simulink model "Six_Step"  (R2023a)
settings: Solver=FixedStepDiscrete  StartTime=0.0  StopTime=SC.T  FixedStep=P.dt  RelTol=1e-3
PreLoadFcn:
  | d_ = fileparts(get_param(bdroot,'FileName')); addpath(d_, fullfile(d_, '..', 'Common')); clear d_; six_step_init;
values from neighbouring files (symbols this model uses):
  DECIM = 10    [six_step_init.m]
  P = bldc_params()    [six_step_init.m]
  SS = struct()    [six_step_init.m]
undefined symbols (not defined in the file or in its folder): THETA_OFF
libraries: bldc_plant_lib x5, slpidlib x2, spspowerguiLib x1
settings Model: Creator=PC  LastModifiedBy=PC

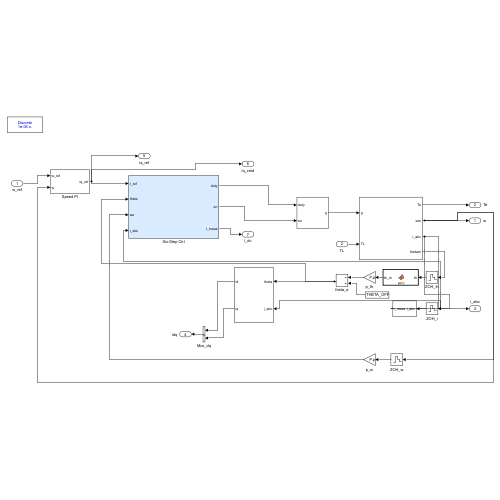
[thumbnail: Simulink's stored preview of the top-level diagram]
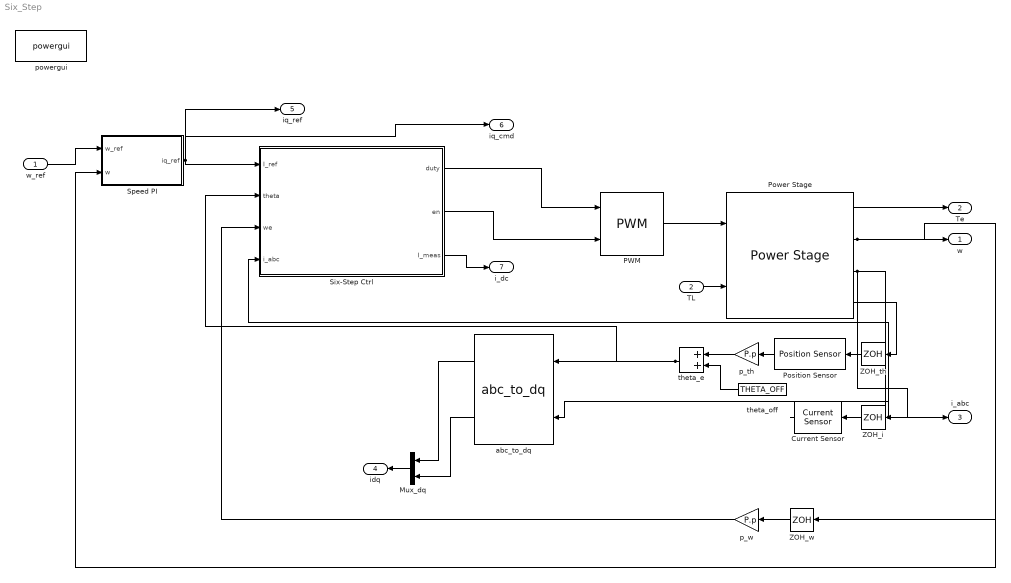
== system Six_Step ==
  w_ref : Inport  Interpolate=off
  TL : Inport  Port=2  Interpolate=off
  Current Sensor : bldc_plant_lib/Current Sensor  Description=Phase-current sensors: i_meas = P.CS.M*(P.CS.gain.*i_abc + P.CS.off). Ideal by default (bldc_set_sensor).  SystemSampleTime=-1  VariantActivationTime=update diagram  Latency=0  AutoFrameSizeCalculation=off
  Mux_dq : Mux  Inputs=2
  PWM : bldc_plant_lib/PWM  SystemSampleTime=-1  VariantActivationTime=update diagram  Latency=0  AutoFrameSizeCalculation=off
  Position Sensor : bldc_plant_lib/Position Sensor  Description=Position sensor: quantized mechanical angle + mounting offset (P.ENC, bldc_set_encoder). Ideal by default.  SystemSampleTime=-1  VariantActivationTime=update diagram  Latency=0  AutoFrameSizeCalculation=off
      settings: LibrarySourceBlock=|
      | simulink/User-Defined
      | Functions/MATLAB Function
  Power Stage : bldc_plant_lib/Power Stage  SystemSampleTime=-1  VariantActivationTime=update diagram  Latency=0  AutoFrameSizeCalculation=off
  Six-Step Ctrl : Subsystem
  Speed PI : Subsystem
  ZOH_i : ZeroOrderHold  SampleTime=P.Ts
  ZOH_th : ZeroOrderHold  SampleTime=P.Ts
  ZOH_w : ZeroOrderHold  SampleTime=P.Ts
  abc_to_dq : bldc_plant_lib/abc_to_dq  SystemSampleTime=-1  VariantActivationTime=update diagram  Latency=0  AutoFrameSizeCalculation=off
  p_th : Gain  Gain=P.p
  p_w : Gain  Gain=P.p
  powergui : spspowerguiLib/powergui  Priority=1  SimulationMode=Discrete  SampleTime=P.dt  frequency=60  Iterations=50  frequencyindice=0  Pbase=100e6  ErrMax=1e-4  UnitsV=kV  UnitsW=MW  buscounter=0  FunctionMessages=off  echomessages=off  EnableUseOfTLC=off  CurrentSourceSwitches=off  DisableSnubberDevices=off  DisableRonSwitches=off  DisableVfSwitches=off  DisplayEquations=off  AutomaticDiscreteSolvers=off  SolverType=Tustin/Backward Euler (TBE)  Interpol=off  ExternalGateDelay=off  methode=off  Ts=100  x0status=blocks  SPID=on  SwTol=0  HookPort=off  NonlinearTolerance=1e-4  nMaxIteration=100  ContinueOnMaxIteration=off  RestoreLinks=warning  ResistiveCurrentMeasurement=off  Frange=[0:2:500]  Ylog=off  Xlog=on  ShowGrid=off  save=off  variable=ZData  structure=0  ZoomFFT=off  StartTime=0.0  cycles=1  DisplayStyle=1  fundamental=60  FreqAxis=off  MaxFrequency=1000  frequencyindicesteady=1  RmsSteady=1  display=off
  theta_e : Sum
  theta_off : Constant  Value=THETA_OFF
  w : Outport  SampleTime=DECIM*P.dt
  Te : Outport  Port=2  SampleTime=DECIM*P.dt
  i_abc : Outport  Port=3  SampleTime=DECIM*P.dt
  idq : Outport  Port=4
  iq_ref : Outport  Port=5
  iq_cmd : Outport  Port=6
  i_dc : Outport  Port=7
  wires:
  w_ref/1 -> Speed PI/1(w_ref)
  Speed PI/1(iq_ref) -> iq_ref/1, Six-Step Ctrl/1(I_ref), iq_cmd/1
  TL/1 -> Power Stage/2
  PWM/1 -> Power Stage/1
  Power Stage/1 -> Te/1
  p_th/1 -> theta_e/1
  theta_off/1 -> theta_e/2
  ZOH_w/1 -> p_w/1
  abc_to_dq/1 -> Mux_dq/1
  abc_to_dq/2 -> Mux_dq/2
  Mux_dq/1 -> idq/1
  Six-Step Ctrl/1(duty) -> PWM/1
  Six-Step Ctrl/2(en) -> PWM/2
  Six-Step Ctrl/3(I_meas) -> i_dc/1
  Power Stage/2 -> w/1, ZOH_w/1, Speed PI/2(w)
  Power Stage/3 -> i_abc/1, ZOH_i/1
  Power Stage/4 -> ZOH_th/1
  theta_e/1 -> abc_to_dq/1, Six-Step Ctrl/2(theta)
  p_w/1 -> Six-Step Ctrl/3(we)
  ZOH_i/1 -> Current Sensor/1
  Current Sensor/1 -> abc_to_dq/2, Six-Step Ctrl/4(i_abc)
  ZOH_th/1 -> Position Sensor/1
  Position Sensor/1 -> p_th/1

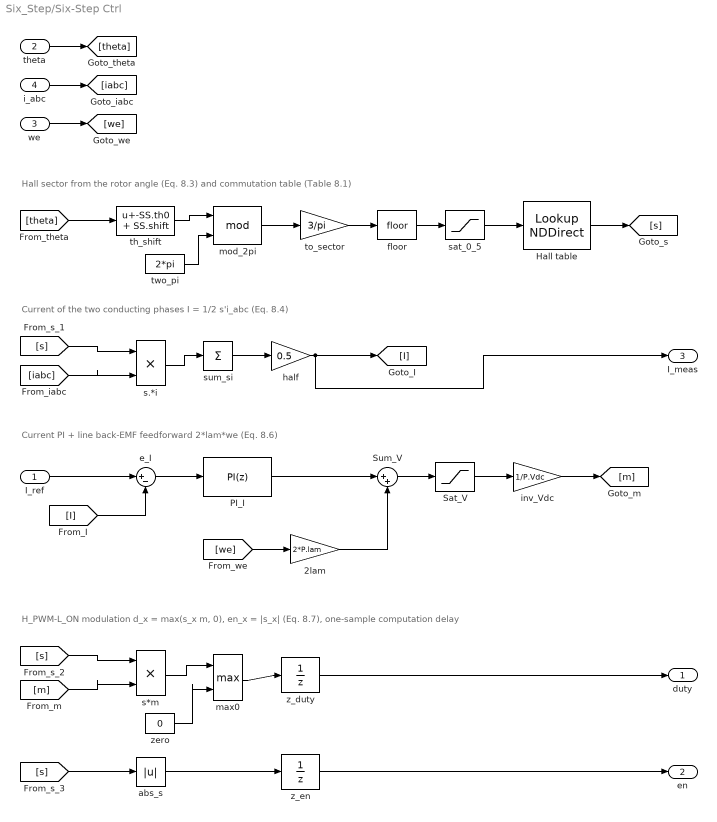
== system Six_Step/Six-Step Ctrl ==
  note: Hall sector from the rotor angle (Eq. 8.3) and commutation table (Table 8.1)
  note: Current of the two conducting phases I = 1/2 s'i_abc (Eq. 8.4)
  note: Current PI + line back-EMF feedforward 2*lam*we (Eq. 8.6)
  note: H_PWM-L_ON modulation d_x = max(s_x m, 0), en_x = |s_x| (Eq. 8.7), one-sample computation delay
  I_ref : Inport
  theta : Inport  Port=2
  we : Inport  Port=3
  i_abc : Inport  Port=4
  2lam : Gain  Gain=2*P.lam
  Hall table : LookupNDDirect  InputsSelectThisObjectFromTable=Vector  Table=SS.tab
  PI_I : slpidlib/PID Controller  Controller=PI  Form=Parallel  TimeDomain=Discrete-time  UseExternalTs=off  SampleTime=P.Ts  IntegratorMethod=Forward Euler  FilterMethod=Forward Euler  ControllerParametersSource=internal  P=P.Kp_i6  I=P.Ki_i6  UseKiTs=off  D=0  N=100  UseFilter=on  TunerSelectOption=Transfer Function Based (PID Tuner App)  InitialConditionSource=internal  InitialConditionForIntegrator=0  InitialConditionForFilter=0  DifferentiatorICPrevScaledInput=0  ExternalReset=none  TrackingMode=off  Kt=1  LimitOutput=on  SatLimitsSource=internal  UpperSaturationLimit=P.Vdc  LowerSaturationLimit=-P.Vdc  LinearizeAsGain=on  AntiWindupMode=back-calculation  Kb=(P.Ki_i6)/(P.Kp_i6)  LimitIntegrator=off  UpperIntegratorSaturationLimit=inf  LowerIntegratorSaturationLimit=-inf  POutMin=[]  POutMax=[]  IOutMin=[]  IOutMax=[]  DOutMin=[]  DOutMax=[]  NOutMin=[]  NOutMax=[]  SumOutMin=[]  SumOutMax=[]  SaturationOutMin=[]  SaturationOutMax=[]  PParamMin=[]  PParamMax=[]  IParamMin=[]  IParamMax=[]  DParamMin=[]  DParamMax=[]  NParamMin=[]  NParamMax=[]  KbParamMin=[]  KbParamMax=[]  KtParamMin=[]  KtParamMax=[]  KbOutMin=[]  KbOutMax=[]  KtOutMin=[]  KtOutMax=[]  IntegratorOutMin=[]  IntegratorOutMax=[]  FilterOutMin=[]  FilterOutMax=[]  SumI1OutMin=[]  SumI1OutMax=[]  SumI2OutMin=[]  SumI2OutMax=[]  SumI3OutMin=[]  SumI3OutMax=[]  SumI4OutMin=[]  SumI4OutMax=[]  SumDOutMin=[]  SumDOutMax=[]  DifferentiatorOutMin=[]  DifferentiatorOutMax=[]  FilterDiffOutCoefMin=[]  FilterDiffOutCoefMax=[]  ReciprocalOutMin=[]  ReciprocalOutMax=[]  SumDenOutMin=[]  SumDenOutMax=[]  SumNumOutMin=[]  SumNumOutMax=[]  DivideOutMin=[]  DivideOutMax=[]  UdiffTsProdOutMin=[]  UdiffTsProdOutMax=[]  NTsProdOutMin=[]  NTsProdOutMax=[]  UintegralTsProdOutMin=[]  UintegralTsProdOutMax=[]  UngainTsProdOutMin=[]  UngainTsProdOutMax=[]  ClampingZeroOutDataTypeStr=Inherit: Inherit via back propagation  ClampingZeroOutMin=[]  ClampingZeroOutMax=[]  FilterDenConstantOutDataTypeStr=Inherit: Inherit via back propagation  FilterDenConstantOutMin=[]  FilterDenConstantOutMax=[]  PCopyOutDataTypeStr=Inherit: Inherit via back propagation  PCopyOutMin=[]  PCopyOutMax=[]  NCopyOutDataTypeStr=Inherit: Inherit via back propagation  NCopyOutMin=[]  NCopyOutMax=[]  IntegratorContinuousStateAttributes=''  IntegratorStateMustResolveToSignalObject=off  IntegratorRTWStateStorageClass=Auto  FilterContinuousStateAttributes=''  FilterStateMustResolveToSignalObject=off  FilterRTWStateStorageClass=Auto  ParallelPVariant=InternalParameters  IdealPVariant=Disabled  IVariant=InternalParameters  DVariant=Disabled  IntegratorVariant=Discrete  SatVariant=Enabled  AWVariant=BackCalculation  PCopyVariant=Disabled  TRVariant=Disabled  FdbkBlocksVariant=Forward  IdealPFdbkVariant=Disabled  SatFdbkVariant=Disabled  DerivativeFilterVariant=Disabled  NVariant=Disabled  NCopyVariant=Disabled_SignalSpec  FilterICVariant=Disabled  IntegratorICVariant=InternalICs  ExternalResetVariant=Disabled  TRSumVariant=Passthrough  SumFdbkVariant=Disabled  SumVariant=Sum_PI  TsampFilterVariant=InternalTs  TsampNgainVariant=Passthrough  TsampIntegralVariant=Disabled_SignalSpec  ExternalSaturationOutDataTypeStr=Inherit: Same as second input
  Sat_V : Saturate  UpperLimit=P.Vdc  LowerLimit=-P.Vdc
  Sum_V : Sum  Inputs=|++
  abs_s : Abs
  e_I : Sum  Inputs=|+-
  floor : Rounding
  half : Gain  Gain=0.5
  inv_Vdc : Gain  Gain=1/P.Vdc
  max0 : MinMax  Function=max  Inputs=2
  mod_2pi : Math  Operator=mod
  s*m : Product
  s.*i : Product
  sat_0_5 : Saturate  UpperLimit=5  LowerLimit=0
  sum_si : Sum  Inputs=+
  th_shift : Bias  Bias=-SS.th0 + SS.shift
  to_sector : Gain  Gain=3/pi
  two_pi : Constant  Value=2*pi
  z_duty : UnitDelay  InitialCondition=zeros(3,1)  SampleTime=P.Ts
  z_en : UnitDelay  InitialCondition=zeros(3,1)  SampleTime=P.Ts
  zero : Constant  Value=0
  duty : Outport
  en : Outport  Port=2
  I_meas : Outport  Port=3
  wires:
  theta/1 -> [theta]
  i_abc/1 -> [iabc]
  we/1 -> [we]
  [theta] -> th_shift/1
  th_shift/1 -> mod_2pi/1
  two_pi/1 -> mod_2pi/2
  mod_2pi/1 -> to_sector/1
  to_sector/1 -> floor/1
  floor/1 -> sat_0_5/1
  sat_0_5/1 -> Hall table/1
  Hall table/1 -> [s]
  [s] -> s.*i/1
  [iabc] -> s.*i/2
  s.*i/1 -> sum_si/1
  sum_si/1 -> half/1
  half/1 -> [I], I_meas/1
  I_ref/1 -> e_I/1
  [I] -> e_I/2
  e_I/1 -> PI_I/1
  PI_I/1 -> Sum_V/1
  [we] -> 2lam/1
  2lam/1 -> Sum_V/2
  Sum_V/1 -> Sat_V/1
  Sat_V/1 -> inv_Vdc/1
  inv_Vdc/1 -> [m]
  [s] -> s*m/1
  [m] -> s*m/2
  s*m/1 -> max0/1
  zero/1 -> max0/2
  max0/1 -> z_duty/1
  z_duty/1 -> duty/1
  [s] -> abs_s/1
  abs_s/1 -> z_en/1
  z_en/1 -> en/1

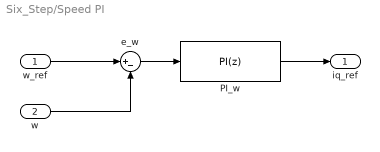
== system Six_Step/Speed PI ==
  w_ref : Inport
  w : Inport  Port=2
  PI_w : slpidlib/PID Controller  Controller=PI  Form=Parallel  TimeDomain=Discrete-time  UseExternalTs=off  SampleTime=P.Tsw  IntegratorMethod=Forward Euler  FilterMethod=Forward Euler  ControllerParametersSource=internal  P=P.Kp_w_6s  I=P.Ki_w_6s  UseKiTs=off  D=0  N=100  UseFilter=on  TunerSelectOption=Transfer Function Based (PID Tuner App)  InitialConditionSource=internal  InitialConditionForIntegrator=0  InitialConditionForFilter=0  DifferentiatorICPrevScaledInput=0  ExternalReset=none  TrackingMode=off  Kt=1  LimitOutput=on  SatLimitsSource=internal  UpperSaturationLimit=P.Imax  LowerSaturationLimit=-P.Imax  LinearizeAsGain=off  AntiWindupMode=back-calculation  Kb=(P.Ki_w_6s)/(P.Kp_w_6s)  LimitIntegrator=off  UpperIntegratorSaturationLimit=inf  LowerIntegratorSaturationLimit=-inf  POutMin=[]  POutMax=[]  IOutMin=[]  IOutMax=[]  DOutMin=[]  DOutMax=[]  NOutMin=[]  NOutMax=[]  SumOutMin=[]  SumOutMax=[]  SaturationOutMin=[]  SaturationOutMax=[]  PParamMin=[]  PParamMax=[]  IParamMin=[]  IParamMax=[]  DParamMin=[]  DParamMax=[]  NParamMin=[]  NParamMax=[]  KbParamMin=[]  KbParamMax=[]  KtParamMin=[]  KtParamMax=[]  KbOutMin=[]  KbOutMax=[]  KtOutMin=[]  KtOutMax=[]  IntegratorOutMin=[]  IntegratorOutMax=[]  FilterOutMin=[]  FilterOutMax=[]  SumI1OutMin=[]  SumI1OutMax=[]  SumI2OutMin=[]  SumI2OutMax=[]  SumI3OutMin=[]  SumI3OutMax=[]  SumI4OutMin=[]  SumI4OutMax=[]  SumDOutMin=[]  SumDOutMax=[]  DifferentiatorOutMin=[]  DifferentiatorOutMax=[]  FilterDiffOutCoefMin=[]  FilterDiffOutCoefMax=[]  ReciprocalOutMin=[]  ReciprocalOutMax=[]  SumDenOutMin=[]  SumDenOutMax=[]  SumNumOutMin=[]  SumNumOutMax=[]  DivideOutMin=[]  DivideOutMax=[]  UdiffTsProdOutMin=[]  UdiffTsProdOutMax=[]  NTsProdOutMin=[]  NTsProdOutMax=[]  UintegralTsProdOutMin=[]  UintegralTsProdOutMax=[]  UngainTsProdOutMin=[]  UngainTsProdOutMax=[]  ClampingZeroOutDataTypeStr=Inherit: Inherit via back propagation  ClampingZeroOutMin=[]  ClampingZeroOutMax=[]  FilterDenConstantOutDataTypeStr=Inherit: Inherit via back propagation  FilterDenConstantOutMin=[]  FilterDenConstantOutMax=[]  PCopyOutDataTypeStr=Inherit: Inherit via back propagation  PCopyOutMin=[]  PCopyOutMax=[]  NCopyOutDataTypeStr=Inherit: Inherit via back propagation  NCopyOutMin=[]  NCopyOutMax=[]  IntegratorContinuousStateAttributes=''  IntegratorStateMustResolveToSignalObject=off  IntegratorRTWStateStorageClass=Auto  FilterContinuousStateAttributes=''  FilterStateMustResolveToSignalObject=off  FilterRTWStateStorageClass=Auto  ParallelPVariant=InternalParameters  IdealPVariant=Disabled  IVariant=InternalParameters  DVariant=Disabled  IntegratorVariant=Discrete  SatVariant=Enabled  AWVariant=BackCalculation  PCopyVariant=Disabled  TRVariant=Disabled  FdbkBlocksVariant=Forward  IdealPFdbkVariant=Disabled  SatFdbkVariant=Disabled  DerivativeFilterVariant=Disabled  NVariant=Disabled  NCopyVariant=Disabled_SignalSpec  FilterICVariant=Disabled  IntegratorICVariant=InternalICs  ExternalResetVariant=Disabled  TRSumVariant=Passthrough  SumFdbkVariant=Disabled  SumVariant=Sum_PI  TsampFilterVariant=InternalTs  TsampNgainVariant=Passthrough  TsampIntegralVariant=Disabled_SignalSpec  ExternalSaturationOutDataTypeStr=Inherit: Same as second input
      settings: LibrarySourceBlock=simulink/Discrete/Discrete PID Controller
  e_w : Sum  Inputs=|+-
  iq_ref : Outport
  wires:
  PI_w/1 -> iq_ref/1
  e_w/1 -> PI_w/1
  w/1 -> e_w/2
  w_ref/1 -> e_w/1
